simulink model "BEV_Thermal_Management"  (R2025a)
settings: Solver=ode23t  StartTime=0  StopTime=765  MaxStep=5  RelTol=1e-3  AbsTol=1e-3
model workspace: external: MATLAB File BEV_Thermal_Management_param.m (data not in the file)
undefined symbols (not defined in the file): Battery, bulb, cabin_doors_conductivity, cabin_duct_area, cabin_glass_conductivity, cabin_roof_conductivity, cabin_T_init, chiller_area_primary, chiller_N_baffles, chiller_N_tubes, chiller_tube_D, chiller_tube_L, chiller_wall_conductivity, chiller_wall_thickness, compressor_rpm_LUT, condenser_air_area_flow, condenser_air_area_primary, condenser_W, condenser_wall_conductivity, condenser_wall_thickness, coolant_channel_D, coolant_pipe_area, coolant_pipe_D, coolant_T_init, coolant_tank_area, coolant_tank_volume, coolant_valve_D_ratio_max, coolant_valve_D_ratio_min, coolant_valve_displacement, coolant_valve_S_max, cycle, DCDC, Edrive, evaporator_air_area_flow, evaporator_air_area_primary, evaporator_W, evaporator_wall_conductivity, evaporator_wall_thickness, heater_max_power, ModuleType1, outlet, ptc_max_power, pump_speed_max, radiationReflectionShields, radiator_air_area_flow, radiator_air_area_primary, radiator_W, radiator_wall_conductivity, radiator_wall_thickness, refrigerant_alpha_init, refrigerant_pipe_D, transRatio
libraries: fl_lib x264, nesl_utility x91, SimscapeFluids_lib x22, sdl_lib x13, ee_lib x9, nesl_utility_internal x4, slpidlib x3, BatteryProtection x3, batt_lib x2, BatteryCurrentManagement x1, autolibsharedcommon x1, simulink x1
(part 9 of 9)

== system BEV_Thermal_Management/Controls/Driver and Regen/Longitudinal Driver ==
  VelRef : Inport  Unit=km/hr
  VelFdbk : Inport  Port=2  Unit=km/hr
  Grade : Inport  Port=3
  AccelHldGround : Ground
  AccelOvrCmdGround : Ground
  AccelZeroGround : Ground
  DecelHldGround : Ground
  DecelOvrCmdGround : Ground
  DecelZeroGround : Ground
  EnblAccelOvrGround : Ground
  EnblDecelOvrGround : Ground
  ExtGearGround : Ground
  External Action Routing : Subsystem
  GearCmdTerminator : Terminator
  Longitudinal Driver : autolibsharedcommon/Longitudinal Driver  cntrlType=PI  shftType=None  vnom=vnom  Kp=Kp  Ki=Ki  Kaw=Kaw  Kff=Kff  Kg=Kg  tauerr=tauerr  tShift=tShift  tRev=tRev  tPark=tPark  pdlVec=pdlVec  upShftTbl=upShftTbl  dwnShftTbl=dwnShftTbl  GearInit=GearInit  tClutch=tClutch  VehVelVec=VehVelVec  KffVec=KffVec  KiVec=KiVec  KpVec=KpVec  KgVec=KgVec  m=m  Kpt=Kpt  Lvv=L  g=g  UpGearVec=UpGearVec  DownGearVec=DownGearVec  aMode=6  errUnit=km/hr  aR=aR  bR=bR  cR=cR  tauPt=tauPt
      settings: LibrarySourceBlock=autolibshared/Longitudinal Driver/Longitudinal Driver
  Info : Outport  InitialOutput=0  VectorParamsAs1DForOutWhenUnconnected=off
  AccelCmd : Outport  Port=2  VectorParamsAs1DForOutWhenUnconnected=off
  DecelCmd : Outport  Port=3  VectorParamsAs1DForOutWhenUnconnected=off
  wires:
  VelRef/1 -> Longitudinal Driver/1
  VelFdbk/1 -> Longitudinal Driver/2
  Longitudinal Driver/1 -> Info/1
  Longitudinal Driver/2 -> AccelCmd/1
  Longitudinal Driver/3 -> DecelCmd/1
  Grade/1 -> Longitudinal Driver/3
  External Action Routing/1(ExtActions) -> Longitudinal Driver/5
  ExtGearGround/1 -> Longitudinal Driver/4
  EnblAccelOvrGround/1 -> External Action Routing/1(EnblAccelOvr)
  AccelOvrCmdGround/1 -> External Action Routing/2(AccelOvrCmd)
  AccelHldGround/1 -> External Action Routing/3(AccelHld)
  AccelZeroGround/1 -> External Action Routing/4(AccelZero)
  EnblDecelOvrGround/1 -> External Action Routing/5(EnblDecelOvr)
  DecelOvrCmdGround/1 -> External Action Routing/6(DecelOvrCmd)
  DecelHldGround/1 -> External Action Routing/7(DecelHld)
  DecelZeroGround/1 -> External Action Routing/8(DecelZero)
  Longitudinal Driver/4 -> GearCmdTerminator/1

== system BEV_Thermal_Management/Controls/Driver and Regen/Regen Braking ==
  note: Copyright 2015-2025 The MathWorks, Inc.
  EMSpd : Inport  OutDataTypeStr=double  PortDimensions=1
  AccelPdl : Inport  Port=2  OutDataTypeStr=double  PortDimensions=1
  DecelCmd : Inport  Port=3  OutDataTypeStr=double
  VehSpdFdbk : Inport  Port=4  OutDataTypeStr=double  PortDimensions=1
  Accel Pedal to Traction Wheel Torque Request : Subsystem  InitFcn=[~]=autosharedicon('autolibinternalvvblock',gcb,0,'6');
  Brake Pedal to Braking Pressure Request : Subsystem
  Motor Torque Arbitration and Power Management : Subsystem
  Regen Braking Control : Subsystem  Commented=on  Variant=on  VariantControlMode=label  VariantControl=(default)  LabelModeActiveChoice=Variant
  Regenerative Braking Logic : Subsystem
  Selector1 : Selector  InputPortWidth=1  IndexOptions=Index vector (dialog)  Indices=[1 1 1 1]  OutputSizes=1
  EMTrqCmd : Outport  OutDataTypeStr=double  PortDimensions=1  VectorParamsAs1DForOutWhenUnconnected=off
  VcuBrkPrsCmd : Outport  Port=2  OutDataTypeStr=double  PortDimensions=4  VectorParamsAs1DForOutWhenUnconnected=off
  wires:
  Accel Pedal to Traction Wheel Torque Request/1(TrqCmd) -> Motor Torque Arbitration and Power Management/1(EMTrqCmdTrac)
  [AccelPdl] -> Motor Torque Arbitration and Power Management/2(AccelPdl)
  Motor Torque Arbitration and Power Management/1(EMTrqCmdFinal) -> EMTrqCmd/1  "EMTrqCmd"
  DecelCmd/1 -> Selector1/1  "DecelPdl"
  [EMSpd] -> Accel Pedal to Traction Wheel Torque Request/2(EMSpd)
  Regenerative Braking Logic/2(" BrkCmd") -> VcuBrkPrsCmd/1  "BrkCmd"
  AccelPdl/1 -> [AccelPdl], Accel Pedal to Traction Wheel Torque Request/1(AccelPdl)
  Regenerative Braking Logic/1(" EMTrqCmdRegen") -> Motor Torque Arbitration and Power Management/3(EMTrqCmdRegen)  "EMTrqCmdRegen"
  EMSpd/1 -> [EMSpd], Regenerative Braking Logic/2("EMSpd ")  "EMSpd"
  Selector1/1 -> Brake Pedal to Braking Pressure Request/1(BcuBrkPrsCmd)  "BrakePrsCmd"
  Brake Pedal to Braking Pressure Request/1(BrkPrsReq) -> Regenerative Braking Logic/3("BrkPrsReq ")
  VehSpdFdbk/1 -> Regenerative Braking Logic/1("VehSpd ")  "VehSpd"

== system BEV_Thermal_Management/Controls/Fan Control/Condenser Requirement ==
  p_cond : Inport
  T_env : Inport  Port=2
  1-D Lookup Table : Lookup_n-D  NumberOfTableDimensions=1  BreakpointsForDimension1=[0 20 30 40 50]  IndexSearchMethod=Linear search  BeginIndexSearchUsingPreviousIndexResult=on  Table=[2.0 2.0 1.8 1.5 1.3]  InternalRulePriority=Speed  RndMeth=Simplest
  1-D Lookup Table1 : Lookup_n-D  NumberOfTableDimensions=1  BreakpointsForDimension1=[0 20 30 40 50]  IndexSearchMethod=Linear search  BeginIndexSearchUsingPreviousIndexResult=on  Table=[1.4 1.4 1.3 1.2 1.1]  InternalRulePriority=Speed  RndMeth=Simplest
  1-D Lookup Table2 : Lookup_n-D  NumberOfTableDimensions=1  BreakpointsForDimension1=[0 20 30 40 50]  IndexSearchMethod=Linear search  BeginIndexSearchUsingPreviousIndexResult=on  Table=[0.8 0.8 0.8 0.8 0.8]  InternalRulePriority=Speed  RndMeth=Simplest
  Bias : Bias  Bias=0.4  SaturateOnIntegerOverflow=off
  Bias1 : Bias  Bias=0.4  SaturateOnIntegerOverflow=off
  Bias2 : Bias  Bias=0.3  SaturateOnIntegerOverflow=off
  Gain : Gain  Gain=1/3
  Relay Level 1 : Subsystem
  Relay Level 2 : Subsystem
  Relay Level 3 : Subsystem
  Sum : Sum  Inputs=+++
  cmd_fan : Outport
  wires:
  Sum/1 -> Gain/1
  p_cond/1 -> Relay Level 3/1(in), Relay Level 2/1(in), Relay Level 1/1(in)
  Relay Level 3/1(out) -> Sum/1
  Relay Level 2/1(out) -> Sum/2
  Relay Level 1/1(out) -> Sum/3
  1-D Lookup Table/1 -> Relay Level 3/3(low), Bias/1
  Bias/1 -> Relay Level 3/2(high)
  1-D Lookup Table1/1 -> Relay Level 2/3(low), Bias1/1
  Bias1/1 -> Relay Level 2/2(high)
  1-D Lookup Table2/1 -> Relay Level 1/3(low), Bias2/1
  Bias2/1 -> Relay Level 1/2(high)
  T_env/1 -> 1-D Lookup Table/1, 1-D Lookup Table1/1, 1-D Lookup Table2/1
  Gain/1 -> cmd_fan/1

== system BEV_Thermal_Management/Controls/Fan Control/Motor Requirement ==
  note: If the motor reaches a temperature above 75°C the fan command is set to its maximum value (which is 1)
  T_motor : Inport
  1-D Lookup Table : Lookup_n-D  NumberOfTableDimensions=1  BreakpointsForDimension1=[-50 45 48 52 58 60 75 130]  IndexSearchMethod=Linear search  BeginIndexSearchUsingPreviousIndexResult=on  Table=[0 0 0.1 0.3 0.5 0.7 1 1]  InternalRulePriority=Speed  RndMeth=Simplest
  cmd_fan : Outport
  wires:
  T_motor/1 -> 1-D Lookup Table/1
  1-D Lookup Table/1 -> cmd_fan/1

== system BEV_Thermal_Management/Scenario/Drive Cycle/Subsystem ==
  VelFdbk : Inport
  Clock : Clock
  Subsystem2 : Subsystem
  Fault : Outport
  UpperBnd : Outport  Port=2
  LowerBnd : Outport  Port=3
  wires:
  Subsystem2/1(upperBound) -> UpperBnd/1  "upperBound"
  VelFdbk/1 -> Subsystem2/2(VelFdbk)
  Clock/1 -> Subsystem2/1(Time)
  Subsystem2/3(faultFlag) -> Fault/1  "Fault"
  Subsystem2/2(lowerBound) -> LowerBnd/1  "lowerBound"

== system BEV_Thermal_Management/Controls/Driver and Regen/Longitudinal Driver/External Action Routing ==
  EnblAccelOvr : Inport  OutDataTypeStr=boolean  Unit=1  PortDimensions=1
  AccelOvrCmd : Inport  Port=2  OutDataTypeStr=double  Unit=1  PortDimensions=1
  AccelHld : Inport  Port=3  OutDataTypeStr=boolean  Unit=1  PortDimensions=1
  AccelZero : Inport  Port=4  OutDataTypeStr=boolean  Unit=1  PortDimensions=1
  EnblDecelOvr : Inport  Port=5  OutDataTypeStr=boolean  Unit=1  PortDimensions=1
  DecelOvrCmd : Inport  Port=6  OutDataTypeStr=double  Unit=1  PortDimensions=1
  DecelHld : Inport  Port=7  OutDataTypeStr=boolean  Unit=1  PortDimensions=1
  DecelZero : Inport  Port=8  OutDataTypeStr=boolean  Unit=1  PortDimensions=1
  Bus Creator2 : BusCreator  Inputs=8
  ExtActions : Outport
  wires:
  EnblAccelOvr/1 -> Bus Creator2/1  "EnblAccelOvr"
  AccelOvrCmd/1 -> Bus Creator2/2  "AccelOvrCmd"
  AccelHld/1 -> Bus Creator2/3  "AccelHld"
  AccelZero/1 -> Bus Creator2/4  "AccelZero"
  EnblDecelOvr/1 -> Bus Creator2/5  "EnblDecelOvr"
  DecelOvrCmd/1 -> Bus Creator2/6  "DecelOvrCmd"
  DecelHld/1 -> Bus Creator2/7  "DecelHld"
  DecelZero/1 -> Bus Creator2/8  "DecelZero"
  Bus Creator2/1 -> ExtActions/1  "ExtActions"

== system BEV_Thermal_Management/Controls/Driver and Regen/Regen Braking/Accel Pedal to Traction Wheel Torque Request ==
  note: Convert Accelerator Pedal Position to Torque Command
      | using Motor Torque Speed Curve
  AccelPdl : Inport
  EMSpd : Inport  Port=2
  MaxEMTrqVsSpd : Lookup_n-D  NumberOfTableDimensions=1  BreakpointsForDimension1=Edrive.torqueCharacteristics.speed  Table=Edrive.torqueCharacteristics.trq  ExtrapMethod=Clip  UseLastTableValue=on  InternalRulePriority=Speed  OutDataTypeStr=Inherit: Inherit from 'Table data'  RndMeth=Simplest
  Product1 : Product
  rads_to_rpm : Gain  Gain=30/pi
  TrqCmd : Outport  VectorParamsAs1DForOutWhenUnconnected=off
  wires:
  Product1/1 -> TrqCmd/1
  MaxEMTrqVsSpd/1 -> Product1/2
  AccelPdl/1 -> Product1/1
  EMSpd/1 -> rads_to_rpm/1
  rads_to_rpm/1 -> MaxEMTrqVsSpd/1

== system BEV_Thermal_Management/Controls/Driver and Regen/Regen Braking/Brake Pedal to Braking Pressure Request ==
  BcuBrkPrsCmd : Inport
  Front Bias : Constant
  Gain4 : Gain  Gain=8000000
  Mux : Mux
  Product : Product
  Rear Bias : Constant  Value=0.6
  BrkPrsReq : Outport  VectorParamsAs1DForOutWhenUnconnected=off
  wires:
  BcuBrkPrsCmd/1 -> Product/2
  Mux/1 -> Product/1
  Rear Bias/1 -> Mux/4, Mux/3
  Front Bias/1 -> Mux/1, Mux/2
  Gain4/1 -> BrkPrsReq/1
  Product/1 -> Gain4/1

== system BEV_Thermal_Management/Controls/Driver and Regen/Regen Braking/Motor Torque Arbitration and Power Management ==
  EMTrqCmdTrac : Inport
  AccelPdl : Inport  Port=2
  EMTrqCmdRegen : Inport  Port=3
  Accel Decel Switch : Switch  Criteria=u2 > Threshold  SaturateOnIntegerOverflow=off  InputSameDT=off
  Compare To Constant : simulink/Logic and Bit Operations/Compare To Constant  relop=>  const=0  OutDataTypeStr=boolean  ZeroCross=off
  EMTrqCmdFinal : Outport  VectorParamsAs1DForOutWhenUnconnected=off
  wires:
  AccelPdl/1 -> Compare To Constant/1
  EMTrqCmdRegen/1 -> Accel Decel Switch/3
  EMTrqCmdTrac/1 -> Accel Decel Switch/1
  Accel Decel Switch/1 -> EMTrqCmdFinal/1
  Compare To Constant/1 -> Accel Decel Switch/2

== system BEV_Thermal_Management/Controls/Driver and Regen/Regen Braking/Regen Braking Control ==
  "VehSpd " : Inport
  "EMSpd " : Inport  Port=2
  "BrkPrsReq " : Inport  Port=3
  Series Regen Braking : Subsystem  InitFcn=[~]=autosharedicon('autolibinternalvvblock',gcb,0,'6');  VariantControl=Variant
  " EMTrqCmdRegen" : Outport  VectorParamsAs1DForOutWhenUnconnected=off
  " BrkCmd" : Outport  Port=2  VectorParamsAs1DForOutWhenUnconnected=off

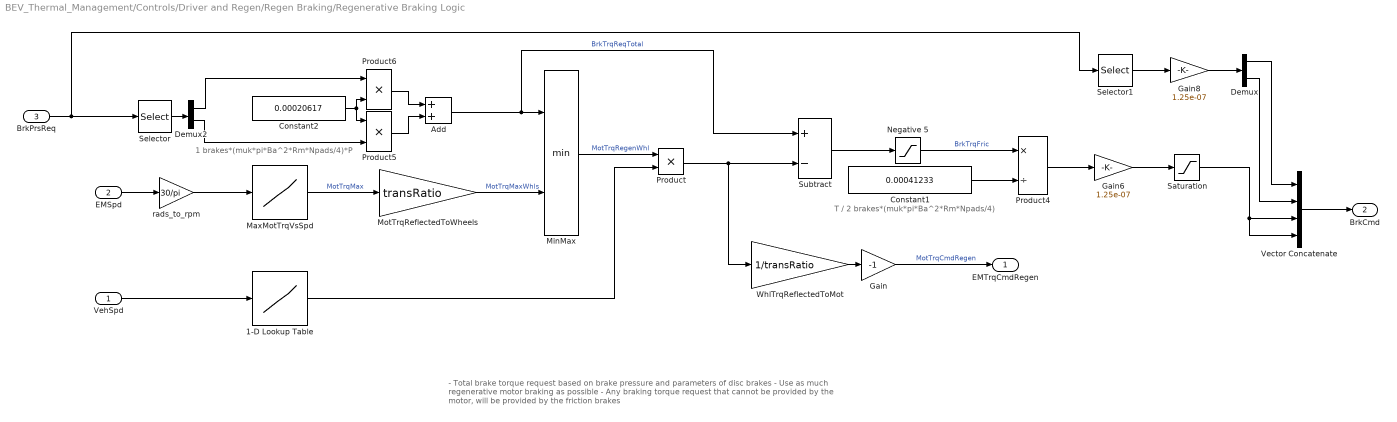
== system BEV_Thermal_Management/Controls/Driver and Regen/Regen Braking/Regenerative Braking Logic ==
  note: T / 2 brakes*(muk*pi*Ba^2*Rm*Npads/4)
  note: - Total brake torque request based on brake pressure and parameters of disc brakes
      | - Use as much regenerative motor braking as possible
      | - Any braking torque request that cannot be provided by the motor, will be provided by the friction brakes
  note: 1 brakes*(muk*pi*Ba^2*Rm*Npads/4)*P
  "VehSpd " : Inport
  "EMSpd " : Inport  Port=2
  "BrkPrsReq " : Inport  Port=3
  1-D Lookup Table : Lookup_n-D  NumberOfTableDimensions=1  BreakpointsForDimension1=[5,9]  Table=[0,1]  ExtrapMethod=Clip  UseLastTableValue=on  InternalRulePriority=Speed  RndMeth=Simplest
  Add : Sum
  Constant1 : Constant  Value=0.00041233
  Constant2 : Constant  Value=0.00020617
  Demux : Demux  Outputs=2
  Demux2 : Demux  Outputs=2
  Gain : Gain  Gain=-1
  Gain6 : Gain  Gain=1.25e-07
  Gain8 : Gain  Gain=1.25e-07
  MaxMotTrqVsSpd : Lookup_n-D  NumberOfTableDimensions=1  BreakpointsForDimension1=Edrive.torqueCharacteristics.speed  Table=Edrive.torqueCharacteristics.trq  ExtrapMethod=Clip  UseLastTableValue=on  InternalRulePriority=Speed  OutDataTypeStr=Inherit: Inherit from 'Table data'  RndMeth=Simplest
  MinMax : MinMax  Inputs=2
  MotTrqReflectedToWheels : Gain  Gain=transRatio
  Negative 5 : Saturate  UpperLimit=inf  LowerLimit=0  ZeroCross=off
  Product : Product
  Product4 : Product  Inputs=*/
  Product5 : Product
  Product6 : Product
  Saturation : Saturate  UpperLimit=1  LowerLimit=0  ZeroCross=off
  Selector : Selector  InputPortWidth=4  IndexOptions=Index vector (dialog)  Indices=[3 4]  OutputSizes=1
  Selector1 : Selector  InputPortWidth=4  IndexOptions=Index vector (dialog)  Indices=[1 2]  OutputSizes=1
  Subtract : Sum  Inputs=+-
  Vector Concatenate : Concatenate  NumInputs=4
  WhlTrqReflectedToMot : Gain  Gain=1/transRatio
  rads_to_rpm : Gain  Gain=30/pi
  " EMTrqCmdRegen" : Outport  VectorParamsAs1DForOutWhenUnconnected=off
  " BrkCmd" : Outport  Port=2  VectorParamsAs1DForOutWhenUnconnected=off
  wires:
  1-D Lookup Table/1 -> Product/2
  Product/1 -> WhlTrqReflectedToMot/1, Subtract/2
  WhlTrqReflectedToMot/1 -> Gain/1
  Selector/1 -> Demux2/1
  Product6/1 -> Add/1
  Demux2/2 -> Product5/2
  Product4/1 -> Gain6/1
  "VehSpd "/1 -> 1-D Lookup Table/1
  Product5/1 -> Add/2
  Selector1/1 -> Gain8/1
  Gain8/1 -> Demux/1
  "BrkPrsReq "/1 -> Selector1/1, Selector/1
  Demux2/1 -> Product6/1
  Gain6/1 -> Saturation/1
  Subtract/1 -> Negative 5/1
  Constant2/1 -> Product5/1, Product6/2
  Negative 5/1 -> Product4/1  "BrkTrqFric"
  rads_to_rpm/1 -> MaxMotTrqVsSpd/1
  "EMSpd "/1 -> rads_to_rpm/1
  MotTrqReflectedToWheels/1 -> MinMax/2  "MotTrqMaxWhls"
  Gain/1 -> " EMTrqCmdRegen"/1  "MotTrqCmdRegen"
  MaxMotTrqVsSpd/1 -> MotTrqReflectedToWheels/1  "MotTrqMax"
  Constant1/1 -> Product4/2
  Add/1 -> Subtract/1, MinMax/1  "BrkTrqReqTotal"
  MinMax/1 -> Product/1  "MotTrqRegenWhl"
  Vector Concatenate/1 -> " BrkCmd"/1
  Saturation/1 -> Vector Concatenate/4, Vector Concatenate/3
  Demux/2 -> Vector Concatenate/2
  Demux/1 -> Vector Concatenate/1

== system BEV_Thermal_Management/Controls/Fan Control/Condenser Requirement/Relay Level 1 ==
  in : Inport
  high : Inport  Port=2
  low : Inport  Port=3
  Data Type Conversion : DataTypeConversion  SaturateOnIntegerOverflow=off  RndMeth=Floor
  Relational Operator : RelationalOperator  OutDataTypeStr=boolean  ZeroCross=off  RndMeth=Simplest  InputSameDT=off
  Relational Operator1 : RelationalOperator  Operator=>  OutDataTypeStr=boolean  ZeroCross=off  RndMeth=Simplest  InputSameDT=off
  Relay : Relay  OnSwitchValue=1.5  OffSwitchValue=0.5
  Sum : Sum  Inputs=|++
  out : Outport
  wires:
  Sum/1 -> Data Type Conversion/1
  Data Type Conversion/1 -> Relay/1
  Relational Operator1/1 -> Sum/2
  Relational Operator/1 -> Sum/1
  Relay/1 -> out/1
  low/1 -> Relational Operator1/2
  high/1 -> Relational Operator/2
  in/1 -> Relational Operator/1, Relational Operator1/1

== system BEV_Thermal_Management/Controls/Fan Control/Condenser Requirement/Relay Level 2 ==
  in : Inport
  high : Inport  Port=2
  low : Inport  Port=3
  Data Type Conversion : DataTypeConversion  SaturateOnIntegerOverflow=off  RndMeth=Floor
  Relational Operator : RelationalOperator  OutDataTypeStr=boolean  ZeroCross=off  RndMeth=Simplest  InputSameDT=off
  Relational Operator1 : RelationalOperator  Operator=>  OutDataTypeStr=boolean  RndMeth=Simplest  InputSameDT=off
  Relay : Relay  OnSwitchValue=1.5  OffSwitchValue=0.5
  Sum : Sum  Inputs=|++
  out : Outport
  wires:
  Sum/1 -> Data Type Conversion/1
  Data Type Conversion/1 -> Relay/1
  Relational Operator1/1 -> Sum/2
  Relational Operator/1 -> Sum/1
  Relay/1 -> out/1
  low/1 -> Relational Operator1/2
  high/1 -> Relational Operator/2
  in/1 -> Relational Operator/1, Relational Operator1/1

== system BEV_Thermal_Management/Controls/Fan Control/Condenser Requirement/Relay Level 3 ==
  in : Inport
  high : Inport  Port=2
  low : Inport  Port=3
  Data Type Conversion : DataTypeConversion  SaturateOnIntegerOverflow=off  RndMeth=Floor
  Relational Operator : RelationalOperator  OutDataTypeStr=boolean  ZeroCross=off  RndMeth=Simplest  InputSameDT=off
  Relational Operator1 : RelationalOperator  Operator=>  OutDataTypeStr=boolean  ZeroCross=off  RndMeth=Simplest  InputSameDT=off
  Relay : Relay  OnSwitchValue=1.5  OffSwitchValue=0.5
  Sum : Sum  Inputs=|++
  out : Outport
  wires:
  Sum/1 -> Data Type Conversion/1
  Data Type Conversion/1 -> Relay/1
  Relational Operator1/1 -> Sum/2
  Relational Operator/1 -> Sum/1
  Relay/1 -> out/1
  low/1 -> Relational Operator1/2
  high/1 -> Relational Operator/2
  in/1 -> Relational Operator/1, Relational Operator1/1

== system BEV_Thermal_Management/Scenario/Drive Cycle/Subsystem/Subsystem2 ==
  Time : Inport
  VelFdbk : Inport  Port=2
  1-D Lookup Table : Lookup_n-D  NumberOfTableDimensions=1  LookupTableObject=''  BreakpointsForDimension1=time  BeginIndexSearchUsingPreviousIndexResult=on  Table=velocity+2  ExtrapMethod=Clip  UseLastTableValue=on  InternalRulePriority=Speed  RndMeth=Simplest
  1-D Lookup Table1 : Lookup_n-D  NumberOfTableDimensions=1  LookupTableObject=''  BreakpointsForDimension1=time  BeginIndexSearchUsingPreviousIndexResult=on  Table=velocity-2  ExtrapMethod=Clip  UseLastTableValue=on  InternalRulePriority=Speed  RndMeth=Simplest
  GreaterThan : RelationalOperator  Operator=>  OutDataTypeStr=boolean  RndMeth=Simplest  InputSameDT=off
  GreaterThan1 : RelationalOperator  Operator=<  OutDataTypeStr=boolean  RndMeth=Simplest  InputSameDT=off
  OR : Logic  Operator=OR  IconShape=distinctive  AllPortsSameDT=off  OutDataTypeStr=boolean
  upperBound : Outport
  lowerBound : Outport  Port=2
  faultFlag : Outport  Port=3
  wires:
  GreaterThan/1 -> OR/1
  1-D Lookup Table/1 -> upperBound/1, GreaterThan/2  "upperBound"
  VelFdbk/1 -> GreaterThan1/1, GreaterThan/1
  Time/1 -> 1-D Lookup Table/1, 1-D Lookup Table1/1
  OR/1 -> faultFlag/1
  GreaterThan1/1 -> OR/2
  1-D Lookup Table1/1 -> lowerBound/1, GreaterThan1/2  "lowerBound"

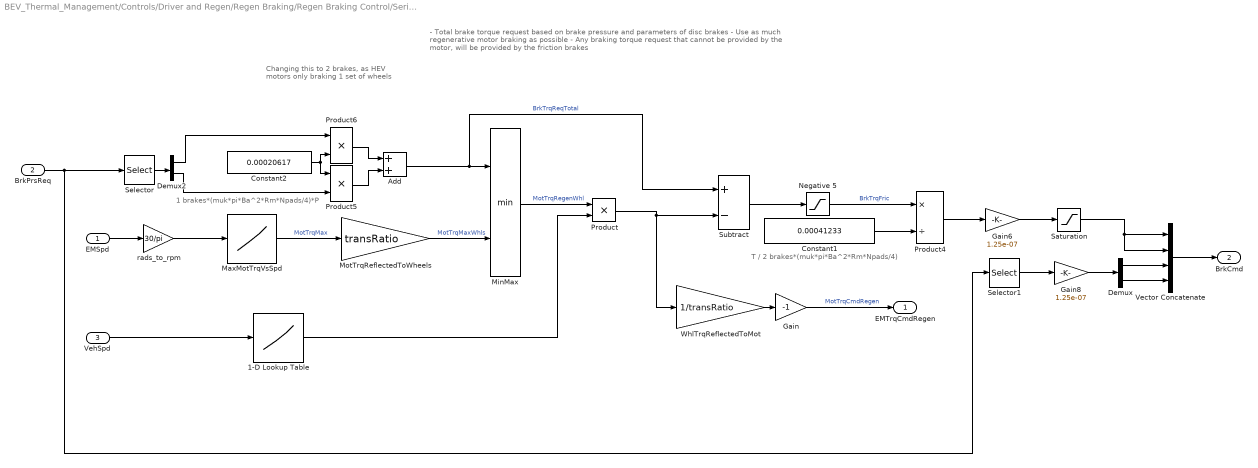
== system BEV_Thermal_Management/Controls/Driver and Regen/Regen Braking/Regen Braking Control/Series Regen Braking ==
  note: - Total brake torque request based on brake pressure and parameters of disc brakes
      | - Use as much regenerative motor braking as possible
      | - Any braking torque request that cannot be provided by the motor, will be provided by the friction brakes
  note: T / 2 brakes*(muk*pi*Ba^2*Rm*Npads/4)
  note: Changing this to 2 brakes,
      | as HEV motors only braking
      | 1 set of wheels
  note: 1 brakes*(muk*pi*Ba^2*Rm*Npads/4)*P
  "EMSpd " : Inport
  "BrkPrsReq " : Inport  Port=2
  "VehSpd " : Inport  Port=3
  1-D Lookup Table : Lookup_n-D  NumberOfTableDimensions=1  BreakpointsForDimension1=[5,9]  Table=[0,1]  InternalRulePriority=Speed  RndMeth=Simplest
  Add : Sum
  Constant1 : Constant  Value=0.00041233
  Constant2 : Constant  Value=0.00020617
  Demux : Demux  Outputs=2
  Demux2 : Demux  Outputs=2
  Gain : Gain  Gain=-1
  Gain6 : Gain  Gain=1.25e-07
  Gain8 : Gain  Gain=1.25e-07
  MaxMotTrqVsSpd : Lookup_n-D  NumberOfTableDimensions=1  BreakpointsForDimension1=Edrive.torqueCharacteristics.speed  Table=Edrive.torqueCharacteristics.trq  ExtrapMethod=Clip  UseLastTableValue=on  InternalRulePriority=Speed  OutDataTypeStr=Inherit: Inherit from 'Table data'  RndMeth=Simplest
  MinMax : MinMax  Inputs=2
  MotTrqReflectedToWheels : Gain  Gain=transRatio
  Negative 5 : Saturate  UpperLimit=inf  LowerLimit=0
  Product : Product
  Product4 : Product  Inputs=*/
  Product5 : Product
  Product6 : Product
  Saturation : Saturate  UpperLimit=1  LowerLimit=0
  Selector : Selector  InputPortWidth=4  IndexOptions=Index vector (dialog)  Indices=[1 2]  OutputSizes=1
  Selector1 : Selector  InputPortWidth=4  IndexOptions=Index vector (dialog)  Indices=[3 4]  OutputSizes=1
  Subtract : Sum  Inputs=+-
  Vector Concatenate : Concatenate  NumInputs=4
  WhlTrqReflectedToMot : Gain  Gain=1/transRatio
  rads_to_rpm : Gain  Gain=30/pi
  " EMTrqCmdRegen" : Outport  VectorParamsAs1DForOutWhenUnconnected=off
  " BrkCmd" : Outport  Port=2  VectorParamsAs1DForOutWhenUnconnected=off
  wires:
  Constant1/1 -> Product4/2
  rads_to_rpm/1 -> MaxMotTrqVsSpd/1
  MaxMotTrqVsSpd/1 -> MotTrqReflectedToWheels/1  "MotTrqMax"
  Subtract/1 -> Negative 5/1
  Negative 5/1 -> Product4/1  "BrkTrqFric"
  "EMSpd "/1 -> rads_to_rpm/1
  MotTrqReflectedToWheels/1 -> MinMax/2  "MotTrqMaxWhls"
  WhlTrqReflectedToMot/1 -> Gain/1
  Gain/1 -> " EMTrqCmdRegen"/1  "MotTrqCmdRegen"
  Demux2/2 -> Product5/2
  Constant2/1 -> Product5/1, Product6/2
  Demux2/1 -> Product6/1
  Selector/1 -> Demux2/1
  Product6/1 -> Add/1
  Product5/1 -> Add/2
  Add/1 -> Subtract/1, MinMax/1  "BrkTrqReqTotal"
  Gain8/1 -> Demux/1
  Saturation/1 -> Vector Concatenate/2, Vector Concatenate/1
  Selector1/1 -> Gain8/1
  "BrkPrsReq "/1 -> Selector1/1, Selector/1
  Vector Concatenate/1 -> " BrkCmd"/1
  Gain6/1 -> Saturation/1
  Demux/1 -> Vector Concatenate/3
  Product4/1 -> Gain6/1
  Demux/2 -> Vector Concatenate/4
  "VehSpd "/1 -> 1-D Lookup Table/1
  1-D Lookup Table/1 -> Product/2
  Product/1 -> WhlTrqReflectedToMot/1, Subtract/2
  MinMax/1 -> Product/1  "MotTrqRegenWhl"
